simulink model "CMSD_Training_Env"  (R2024b)
settings: Solver=VariableStepAuto  StartTime=0.0  StopTime=inf  RelTol=1e-3
undefined symbols (not defined in the file or in its folder): ref_seed
libraries: simulink x1, rllib x1
settings Model: Creator=minhh  LastModifiedBy=minhh
settings DebuggingCC: SignalInfNanChecking=error

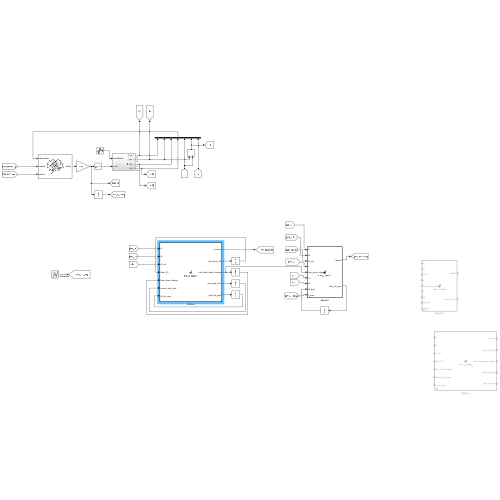
[thumbnail: Simulink's stored preview of the top-level diagram]
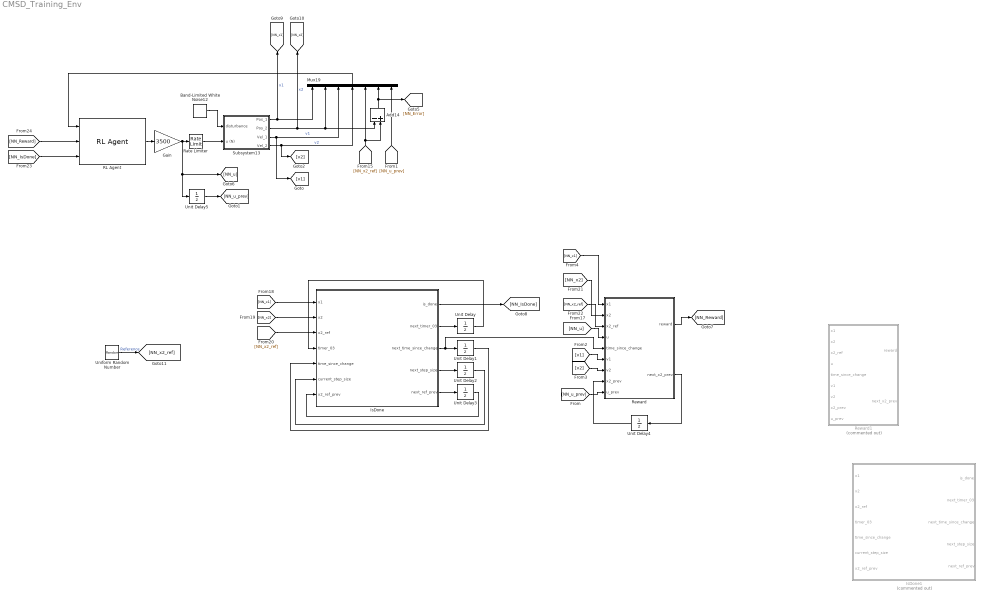
== system CMSD_Training_Env ==
  Add14 : Sum  Inputs=-+
  Band-Limited White Noise12 : simulink/Sources/Band-Limited White Noise  Cov=[200]  Ts=0.01  seed=noise_seed
  Gain : Gain  Gain=3500
  IsDone : MATLAB Function  TreatAsAtomicUnit=on
  IsDone1 : MATLAB Function  Commented=on  TreatAsAtomicUnit=on
  Mux19 : Mux  Inputs=7
  RL Agent : rllib/RL Agent  Agent=agentObj  ExternalActionAsInput=off  ProvideLastAction=off  ProvideCumRwd=off  TreatAsDirectFeedthrough=on  UseStrictObservationDataTypes=off
  Rate Limiter : RateLimiter  RisingSlewLimit=25000  FallingSlewLimit=-25000  SampleTimeMode=inherited
  Reward : MATLAB Function  TreatAsAtomicUnit=on
  Reward1 : MATLAB Function  Commented=on  TreatAsAtomicUnit=on
  Subsystem13 : Subsystem
  Uniform Random Number : UniformRandomNumber  Minimum=0  Maximum=0.5  Seed=ref_seed  SampleTime=30
  Unit Delay{,1..5} (6 alike) : UnitDelay  SampleTime=0.01  HasFrameUpgradeWarning=on
  wires:
  [NN_x2_ref] -> IsDone/3(x2_ref)
  Uniform Random Number/1 -> [NN_x2_ref]  "Reference"
  IsDone/5(next_ref_prev) -> Unit Delay3/1
  Unit Delay/1 -> IsDone/4(timer_03)
  [NN_x2_ref] -> Reward/3(x2_ref)
  IsDone/2(next_timer_03) -> Unit Delay/1
  Unit Delay1/1 -> IsDone/5(time_since_change)
  [NN_x1] -> IsDone/1(x1)
  Unit Delay2/1 -> IsDone/6(current_step_size)
  [NN_x2] -> IsDone/2(x2)
  Add14/1 -> [NN_Error], Mux19/6
  Reward/2(next_x2_prev) -> Unit Delay4/1
  Unit Delay3/1 -> IsDone/7(x2_ref_prev)
  [NN_u] -> Reward/4(u)
  [NN_Reward] -> RL Agent/2
  Unit Delay4/1 -> Reward/8(x2_prev)
  Rate Limiter/1 -> Subsystem13/2(u (N))
  IsDone/4(next_step_size) -> Unit Delay2/1
  [NN_x2_ref] -> Mux19/5, Add14/2
  IsDone/1(is_done) -> [NN_IsDone]
  Band-Limited White Noise12/1 -> Subsystem13/1(disturbance)
  Reward/1(reward) -> [NN_Reward]
  Subsystem13/4(Vel_2) -> [v2], Mux19/4  "v2"
  [NN_x2] -> Reward/2(x2)
  Subsystem13/1(Pos_1) -> Mux19/1, [NN_x1]  "x1"
  [NN_IsDone] -> RL Agent/3
  Subsystem13/2(Pos_2) -> Add14/1, Mux19/2, [NN_x2]  "x2"
  IsDone/3(next_time_since_change) -> Reward/5(time_since_change), Unit Delay1/1
  Subsystem13/3(Vel_1) -> [v1], Mux19/3  "v1"
  RL Agent/1 -> Gain/1
  [NN_u_prev] -> Reward/9(u_prev)
  Gain/1 -> Unit Delay5/1, [NN_u], Rate Limiter/1
  Unit Delay5/1 -> [NN_u_prev]
  [NN_u_prev] -> Mux19/7
  Mux19/1 -> RL Agent/1
  [v1] -> Reward/6(v1)
  [v2] -> Reward/7(v2)
  [NN_x1] -> Reward/1(x1)

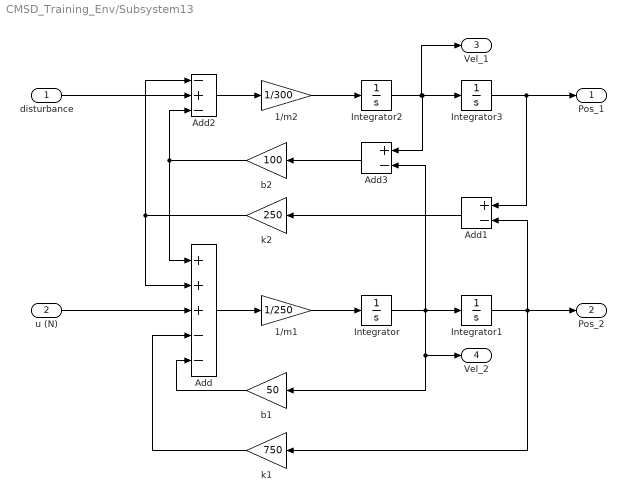
== system CMSD_Training_Env/Subsystem13 ==
  disturbance : Inport
  u (N) : Inport  Port=2
  1/m1 : Gain  Gain=1/250
  1/m2 : Gain  Gain=1/300
  Add : Sum  Inputs=+++--
  Add1 : Sum  Inputs=+-
  Add2 : Sum  Inputs=-+-
  Add3 : Sum  Inputs=+-
  Integrator{,1..3} (4 alike) : Integrator
  b1 : Gain  Gain=50
  b2 : Gain  Gain=100
  k1 : Gain  Gain=750
  k2 : Gain  Gain=250
  Pos_1 : Outport
  Pos_2 : Outport  Port=2
  Vel_1 : Outport  Port=3
  Vel_2 : Outport  Port=4
  wires:
  Add/1 -> 1/m1/1
  1/m1/1 -> Integrator/1
  Integrator/1 -> Add3/2, Integrator1/1, b1/1, Vel_2/1
  Integrator1/1 -> k1/1, Pos_2/1, Add1/2
  Add2/1 -> 1/m2/1
  1/m2/1 -> Integrator2/1
  Integrator2/1 -> Vel_1/1, Add3/1, Integrator3/1
  Add3/1 -> b2/1
  b2/1 -> Add2/3, Add/1
  Add1/1 -> k2/1
  Integrator3/1 -> Pos_1/1, Add1/1
  u (N)/1 -> Add/3
  b1/1 -> Add/5
  k1/1 -> Add/4
  k2/1 -> Add2/1, Add/2
  disturbance/1 -> Add2/2

== matlab function CMSD_Training_Env/Reward1 ==
  data: x1 input; x2 input; x2_ref input; u input; time_since_change input; v1 input; v2 input; reward output; x2_prev input; next_x2_prev output; u_prev input
function [reward, next_x2_prev] = calc_reward(x1, x2, x2_ref, u, time_since_change, v1, v2, x2_prev, u_prev)

% =========================================================================
% calc_reward.m — CMSD NN Controller Reward Function
%
% Argument order (must match Simulink block wiring):
%   x2, x2_ref, u, time_since_change, v1, v2, x2_prev, u_prev
%
% Key changes from previous version:
%   - violation^2 replaced with linear penalty  → fixes billion-reward bug
%   - per-step hard floor at -20                → agent always gets signal
%   - energy term scaled down (was dominating)  → u^2 → 0.01*(u/3500)^2
%   - v2 check uses abs(v2) (was unsigned)      → catches oscillation both ways
%   - all reward components kept proportional   → good ep ≈ +2000, bad ≈ -15000
% =========================================================================

% --- ENFORCE STRICT DATA TYPES FOR COMPILER ---
    reward       = double(0.1);
    next_x2_prev = double(x2);
    x2_error     = double(abs(x2_ref - x2));
    delta_u      = double(abs(u - u_prev));   % u is post-gain (Newtons)

% --- 1. TRACKING — primary goal (your original weights kept) ---
    reward = double(reward - (10.0 * x2_error^2));

% --- 2. TIGHT ZONE BONUS / MISS PENALTY ---
%   Your original ±1/+2 split kept, just clarified
    if x2_error < 0.01
        reward = double(reward + 2.0);    % inside 10mm — excellent
    elseif x2_error < 0.050
        reward = double(reward + 0.5);    % inside 50mm — acceptable
    else
        reward = double(reward - 1.0);    % outside — penalise
    end

% --- 3. SMC ROBUSTNESS — penalise oscillation after settling ---
%   abs(v2) catches oscillation in both directions (your version missed negative v2)
    if time_since_change > 1.0
        if abs(v2) > 0.01
            reward = double(reward - 5.0);
        end
    end

% --- 4. ENERGY EFFICIENCY ---
%   Scaled down from 0.5*(u/3500)^2 to 0.01*(u/3500)^2
%   Original was subtracting up to -0.5 per step just for moving — too aggressive
%   for early training where the agent NEEDS to move to explore.
%   At full force: 0.01 * 1^2 = -0.01 per step (negligible vs tracking signal)
    reward = double(reward - 0.01 * (u / 3500.0)^2);

% --- 5. HARDWARE LIMIT PENALTY — LINEAR, not squared ---
%   FIX: violation^2 was the billion-reward bug.
%   With gain=3500 and random actions, delta_u can reach 7000 N/step.
%   violation = 6500  →  violation^2 = 42,250,000 per step × 1500 steps = -63 billion.
%   Linear version: same signal to the agent (big jumps = bad) without explosion.
%   At worst case: -0.005 * 6500 = -32.5 per step — meaningful but survivable.
    if delta_u > 500.0
        violation = double(delta_u - 500.0);
        reward    = double(reward - (0.005 * violation));   % LINEAR — not squared
    end

% --- 6. VELOCITY DAMPING (your original weights kept) ---
    v1_penalty = double(abs(v1) * 0.02);
    v2_penalty = double(abs(v2) * 0.10);
    reward     = double(reward - v1_penalty - v2_penalty);

% --- 7. PER-STEP HARD FLOOR ---
%   Prevents any single catastrophic step from making the episode reward
%   so negative that the gradient update is meaningless noise.
%   Worst case episode: -20 * 1500 steps = -30,000  (was -2,315,943,825)
    reward = double(max(reward, -20.0));


        % --- THE ANTI-SUICIDE PATCH ---
    % If the AI violently jerks the motor and breaks the x1 limit, 
    % it receives a penalty so massive it will never do it again.
    if abs(x1) > 0.65
        reward = double(reward - 6000.0);
    end


end

== matlab function CMSD_Training_Env/IsDone1 ==
  data: x1 input; is_done output; x2 input; x2_ref input; next_timer_03 output; timer_03 input; time_since_change input; current_step_size input; x2_ref_prev input; next_time_since_change output; next_step_size output; next_ref_prev output
function [is_done, next_timer_03, next_time_since_change, next_step_size, next_ref_prev] = check_safety(x1, x2, x2_ref, timer_03, time_since_change, current_step_size, x2_ref_prev)
    
    % --- ENFORCE STRICT DATA TYPES FOR THE COMPILER ---
    is_done = double(0); % <--- Changed to double(0) instead of false
    next_timer_03 = double(timer_03);
    next_time_since_change = double(time_since_change);
    next_step_size = double(current_step_size);
    next_ref_prev = double(x2_ref_prev);
    
    dt = double(0.01); 
    x2_error = double(x2_ref - x2);
    
    % --- 1. DETECT A REFERENCE CHANGE ---
    if abs(x2_ref - x2_ref_prev) > 0.001
        next_time_since_change = double(0.0);
        next_step_size = double(abs(x2_ref - x2_ref_prev));
    else
        next_time_since_change = double(time_since_change + dt);
    end
    next_ref_prev = double(x2_ref);
    
    % --- 2. DEATH CONDITIONS ---
    if abs(x1) > 0.65
        is_done = double(1); % <--- Changed to double(1) instead of true
    end
    
    if abs(x2_error) > 0.3
        next_timer_03 = double(timer_03 + dt);
    else
        next_timer_03 = double(0.0);
    end
    
    if next_timer_03 > 3.0 % <--- CHANGED TO 3.0 from 0.75
        is_done = double(1); % <--- Changed to double(1)
    end
    
    %if next_step_size > 0
    %    allowed_settle_time = double(next_step_size * 2.2);
    %else
    %    allowed_settle_time = double(2.0); 
    %end


    %=====> RELAXED: Give it a flat 5.0 seconds to settle, regardless of step size
    allowed_settle_time = double(5.0); % <--- BYPASS THE MULTIPLIER FOR NOW

    % Widen the survival boundary to 0.05m (50mm) for early training
    if (next_time_since_change > allowed_settle_time) && (abs(x2_error) > 0.050)
        is_done = double(1); % <--- Changed to double(1)
    end
end

== matlab function CMSD_Training_Env/Reward ==
  data: x1 input; x2 input; x2_ref input; u input; time_since_change input; v1 input; v2 input; reward output; x2_prev input; next_x2_prev output; u_prev input
function [reward, next_x2_prev] = calc_reward(x1, x2, x2_ref, u, time_since_change, v1, v2, x2_prev, u_prev)

% =========================================================================
% calc_reward.m — CMSD NN Controller Reward Function (v5)
%
% Root cause fix: dying fast was more profitable than surviving.
% Per-step cost (-2.48) exceeded per-step income (+0.1) when tracking
% was poor, so the agent rationally chose quick death over long survival.
%
% Fix: base reward raised to +1.0, progress bonus widened so it pays out
% even at 0.3m error, miss penalties removed (quadratic handles distance).
% Now every step alive is net positive, tracking well is 7x better than
% tracking poorly, and dying is always worse than surviving.
%
% Per-step economics (v5):
%   Poor tracking (error=0.3m): +1.0 + 0.64 - 0.9 = +0.74/step (net positive)
%   Good tracking (error=0.01m): +1.0 + 1.0 + 3.0 - 0.001 = +4.99/step
%   Perfect tracking (error=0):  +5.0/step
%   6000-step perfect episode:   ~+30,000 total
% =========================================================================

% --- DATA TYPES ---
    reward       = double(1.0);           % raised from 0.1 — survival has inherent value
    next_x2_prev = double(x2);
    x2_error     = double(abs(x2_ref - x2));
    delta_u      = double(abs(u - u_prev));
    x1_abs       = double(abs(x1));

% --- 1. TRACKING — primary goal ---
%   Quadratic penalty. At error=0.3m: -0.9. At error=1.0m: -10.
%   Kept unchanged — this is the core learning signal.
    reward = double(reward - (10.0 * x2_error^2));

% --- 2. ZONE BONUS (penalties removed) ---
%   Previous version penalised being far from target on top of the
%   quadratic. This double-penalised poor tracking and made per-step cost
%   exceed per-step income, incentivising fast death.
%   Now: bonuses only. Being far costs only through the quadratic term.
    if x2_error < 0.010
        reward = double(reward + 3.0);    % inside 10mm  — excellent
    elseif x2_error < 0.050
        reward = double(reward + 1.5);    % inside 50mm  — good
    elseif x2_error < 0.150
        reward = double(reward + 0.3);    % inside 150mm — acceptable, small bonus
    % No penalty beyond 150mm — quadratic term handles it
    end

% --- 3. PROGRESS / SURVIVAL BONUS ---
%   Widened Gaussian (sigma doubled: -20 -> -5) so bonus pays even at 0.3m.
%   This is what makes every step alive net positive regardless of tracking.
%   At error=0.0m:  +1.0/step (excellent, doubles the base survival reward)
%   At error=0.1m:  +0.95/step (still very good)
%   At error=0.3m:  +0.64/step (meaningful — agent wants to stay alive)
%   At error=1.0m:  +0.007/step (essentially zero — must track to benefit)
    progress_bonus = double(1.0 * exp(-5.0 * x2_error^2));
    reward = double(reward + progress_bonus);

% --- 4. VELOCITY DAMPING after settling ---
%   Only after 1s grace period following reference change.
    if time_since_change > 1.0
        if abs(v2) > 0.05
            reward = double(reward - 1.0);
        end
        if abs(v1) > 0.05
            reward = double(reward - 0.5);
        end
    end

% --- 5. ENERGY EFFICIENCY ---
%   Very small — tiebreaker only, does not dominate learning signal.
    reward = double(reward - 0.01 * (u / 3500.0)^2);

% --- 6. HARDWARE JERK PENALTY — LINEAR ---
    if delta_u > 500.0
        violation = double(delta_u - 500.0);
        reward    = double(reward - (0.005 * violation));
    end

% --- 7. X1 SOFT BARRIER ---
%   Zone-1 from 0.30m, Zone-2 from 0.45m.
%   At x1=0.65m: total ~-1.46/step — costly but not overwhelming.
%   Terminal -500 makes wall approach unambiguously fatal.
    if x1_abs > 0.30
        x1_margin1 = double(x1_abs - 0.30);
        reward = double(reward - (8.0 * x1_margin1^2));
    end
    if x1_abs > 0.45
        x1_margin2 = double(x1_abs - 0.45);
        reward = double(reward - (12.0 * x1_margin2^2));
    end

% --- 8. X1 CENTERING BONUS ---
%   Continuous pull toward x1=0. +0.30/step at centre, fades beyond 0.40m.
    x1_centre_bonus = double(0.30 * exp(-10.0 * x1^2));
    reward = double(reward + x1_centre_bonus);

% --- 9. X1 TERMINAL PENALTY ---
    if x1_abs > 0.65
        reward = double(reward - 500.0);
    end

% --- 10. PER-STEP HARD FLOOR ---
%   Still needed for jerk/barrier spikes. -50 allows large penalties
%   without gradient-destroying billion-scale values.
    reward = double(max(reward, -50.0));

end

== matlab function CMSD_Training_Env/IsDone ==
  data: x1 input; is_done output; x2 input; x2_ref input; next_timer_03 output; timer_03 input; time_since_change input; current_step_size input; x2_ref_prev input; next_time_since_change output; next_step_size output; next_ref_prev output
function [is_done, next_timer_03, next_time_since_change, next_step_size, next_ref_prev] = check_safety(x1, x2, x2_ref, timer_03, time_since_change, current_step_size, x2_ref_prev)

% =========================================================================
% check_safety.m — CMSD Episode Termination (v2)
%
% Changes from v1:
%   - Settle timeout is now PROPORTIONAL to step size (was flat 8.0s)
%     Flat 8s allowed the agent to idle on small steps, contributing to
%     the "do nothing and survive" local minimum seen at episode 150.
%   - x2 error timer threshold widened to 0.5m (kept from v1)
%   - All fprintf diagnostics kept — remove when no longer needed
% =========================================================================

% --- DATA TYPES ---
    is_done                = double(0);
    next_timer_03          = double(timer_03);
    next_time_since_change = double(time_since_change);
    next_step_size         = double(current_step_size);
    next_ref_prev          = double(x2_ref_prev);
    dt                     = double(0.01);
    x2_error               = double(x2_ref - x2);

% --- 1. REFERENCE CHANGE DETECTION ---
    if abs(x2_ref - x2_ref_prev) > 0.001
        next_time_since_change = double(0.0);
        next_step_size         = double(abs(x2_ref - x2_ref_prev));
    else
        next_time_since_change = double(time_since_change + dt);
    end
    next_ref_prev = double(x2_ref);

% --- 2. DEATH A: x1 hard wall ---
    if abs(x1) > 0.65
        is_done = double(1);
        fprintf('DEATH: x1 wall at x1=%.3f\n', x1);
    end

% --- 3. DEATH B: x2 error timer ---
%   Threshold 0.5m — wide enough that normal transients don't trigger it.
%   3 second timer — recycles a completely lost agent quickly.
    error_threshold = double(0.5);
    timer_duration  = double(3.0);

    if abs(x2_error) > error_threshold
        next_timer_03 = double(timer_03 + dt);
    else
        next_timer_03 = double(0.0);
    end

    if next_timer_03 > timer_duration
        is_done = double(1);
        fprintf('DEATH: x2 error timer at x2_err=%.3f\n', abs(x2_error));
    end

% --- 4. DEATH C: settle-time (PROPORTIONAL to step size) ---
%   Flat 8.0s was allowing the agent to idle on small reference steps.
%   A 0.05m step should settle in ~2s. A 1.5m step may need 6s.
%   Formula: max(3.0s minimum, step_size * 4.0 seconds/metre)
%   Examples:
%     step = 0.10m  →  allowed = max(3.0, 0.40) = 3.0s
%     step = 0.50m  →  allowed = max(3.0, 2.00) = 3.0s
%     step = 0.80m  →  allowed = max(3.0, 3.20) = 3.2s
%     step = 1.50m  →  allowed = max(3.0, 6.00) = 6.0s
%   Error band: 50mm — tighten to 30mm once agent survives 1000+ steps
    if next_step_size > 0
        allowed_settle_time = double(max(3.0, next_step_size * 4.0));
    else
        allowed_settle_time = double(3.0);
    end
    error_band = double(0.050);

    if (next_time_since_change > allowed_settle_time) && (abs(x2_error) > error_band)
        is_done = double(1);
        fprintf('DEATH: settle timeout, err=%.3f after %.1fs (allowed=%.1fs)\n', ...
            abs(x2_error), next_time_since_change, allowed_settle_time);
        fprintf('\nx2=%.3f', x2)
    end

end
